simulink model "turbo_controller"  (R2025a)
settings: Solver=FixedStepAuto  StartTime=0.0  StopTime=inf  FixedStep=0.001  RelTol=1e-3
PostLoadFcn:
  | % 自动定位同目录CubeMX文件；不需要外部初始化脚本。
  | codertarget.data.setParameterValue('turbo_controller','STM32CubeMX.ProjectFile',fullfile(fileparts(get_param('turbo_controller','FileName')),'turbo_f407.ioc'));
InitFcn:
  | % 中文说明：按原控制器字段与类型创建三组接口总线；控制参数已内嵌。
  | tc_names=["EValve_Cycle" "EValve_Open" "Eblast_Cycle" "Eblast_Open" "Motor_Cycle" "Motor_Open" "EValve_Enable" "Eblast_Enable" "Motor_Enable" "SWO_Firework" "SWO_BleedAir" "EngineState" "Flag_ECUReset_Clear" "Flag_ECUReset_Save" "Flag_Reset_Enable" "Accelerator" "Nc_dem" "Nc"]; tc_types=["uint16" "uint16" "uint16" "uint16" "uint16" "uint16" "uint8" "uint8" "uint8" "uint8" "uint8" "uint8" "uint8" "uint8" "uint8" "single" "single" "single"];
  | for tc_k=1:numel(tc_names)
  |  tc_e(tc_k)=Simulink.BusElement; tc_e(tc_k).Name=char(tc_names(tc_k)); tc_e(tc_k).DataType=char(tc_types(tc_k));
  | end
  | EngineControl_Out=Simulink.Bus; EngineControl_Out.DataScope='Exported'; EngineControl_Out.Elements=tc_e;
  | clear tc_e tc_names tc_types tc_k
  | tc_names=["savedata1" "savedata2" "savedata3" "savedata4" "savedata5" "savedata6" "savedata7" "savedata8" "savedata9" "savedata10" "savedata11" "savedata12" "savedata13" "savedata14" "savedata15" "savedata16" "savedata17" "savedata18" "savedata19" "savedata20" "savedata21" "savedata22" "savedata23" "savedata24" "savedata25"]; tc_types=["single" "single" "single" "single" "single" "single" "single" "single" "single" "single" "single" "single" "single" "single" "single" "single" "single" "single" "single" "single" "single" "single" "single" "single" "single"];
  | for tc_k=1:numel(tc_names)
  |  tc_e(tc_k)=Simulink.BusElement; tc_e(tc_k).Name=char(tc_names(tc_k)); tc_e(tc_k).DataType=char(tc_types(tc_k));
  | end
  | SaveData_Out=Simulink.Bus; SaveData_Out.DataScope='Exported'; SaveData_Out.Elements=tc_e;
  | clear tc_e tc_names tc_types tc_k
  | tc_names=["senddata1" "senddata2" "senddata3" "senddata4" "senddata5" "senddata6" "senddata7" "senddata8" "senddata9" "senddata10" "senddata11" "senddata12" "senddata13" "senddata14" "senddata15" "senddata16" "senddata17" "senddata18" "senddata19" "senddata20" "senddata21" "senddata22" "senddata23" "senddata24" "senddata25" "senddata26" "senddata27" "senddata28" "senddata29"]; tc_types=["uint8" "uint8" "uint8" "uint8" "uint8" "uint8" "uint8" "uint8" "uint8" "uint8" "uint8" "uint8" "uint8" "uint8" "uint8" "uint8" "uint8" "uint8" "uint8" "uint8" "uint8" "uint8" "uint8" "uint8" "uint8" "uint8" "uint8" "uint8" "uint8"];
  | for tc_k=1:numel(tc_names)
  |  tc_e(tc_k)=Simulink.BusElement; tc_e(tc_k).Name=char(tc_names(tc_k)); tc_e(tc_k).DataType=char(tc_types(tc_k));
  | end
  | SendData_Out=Simulink.Bus; SendData_Out.DataScope='Exported'; SendData_Out.Elements=tc_e;
  | clear tc_e tc_names tc_types tc_k
  | 
  | % 以下为接口中文说明；只设置描述，不改变数值或数据类型。
  | EngineControl_Out.Description='执行控制输出（阀、电机、点火、状态及复位请求）';
  | tc_cn=["EValve_Cycle（主油阀周期计数（每计数2毫秒））" "EValve_Open（主油阀开通计数（每计数2毫秒））" "Eblast_Cycle（副油阀周期计数（每计数2毫秒））" "Eblast_Open（副油阀开通计数（每计数2毫秒））" "Motor_Cycle（起动电机周期计数）" "Motor_Open（起动电机开通计数）" "EValve_Enable（主油阀驱动使能）" "Eblast_Enable（副油阀驱动使能）" "Motor_Enable（起动电机使能）" "SWO_Firework（点火器使能（1开））" "SWO_BleedAir（引气阀使能（1开））" "EngineState（发动机状态）" "Flag_ECUReset_Clear（清除复位恢复状态请求）" "Flag_ECUReset_Save（保存复位恢复数据请求）" "Flag_Reset_Enable（处理器软件复位请求）" "Accelerator（油门／油泵给定控制量）" "Nc_dem（控制目标转速）" "Nc（发动机反馈转速（转每分））"];
  | tc_elements=EngineControl_Out.Elements;
  | for tc_k=1:numel(tc_cn)
  |  tc_elements(tc_k).Description=char(tc_cn(tc_k));
  | end
  | EngineControl_Out.Elements=tc_elements;
  | clear tc_cn tc_elements tc_k
  | SaveData_Out.Description='25项运行记录；字段含义按当前模型数据来源解释';
  | tc_cn=["savedata1（指令回显记录）" "savedata2（入口总温记录（℃））" "savedata3（电源电压记录）" "savedata4（排气温度记录（℃））" "savedata5（标定燃油压力记录）" "savedata6（副油阀占空比记录（％））" "savedata7（主油阀占空比记录（％））" "savedata8（温度修正转速记录）" "savedata9（开关输出及反馈位域）" "savedata10（物理转速记录）" "savedata11（油泵目标给定原始值）" "savedata12（起动电机占空比记录（％））" "savedata13（发动机状态码记录）" "savedata14（故障告警位域记录）" "savedata15（模型记录帧序号）" "savedata16（处理器温度记录（℃））" "savedata17（装订转速记录（沿用旧电源字段名））" "savedata18（导航高度记录）" "savedata19（飞行空速记录）" "savedata20（主阀旧记录位（恒零保留））" "savedata21（第21项保留记录（恒零））" "savedata22（保留记录项22）" "savedata23（保留记录项23）" "savedata24（保留记录项24）" "savedata25（保留记录项25）"];
  | tc_elements=SaveData_Out.Elements;
  | for tc_k=1:numel(tc_cn)
  |  tc_elements(tc_k).Description=char(tc_cn(tc_k));
  | end
  | SaveData_Out.Elements=tc_elements;
  | clear tc_cn tc_elements tc_k
  | SendData_Out.Description='29字段回传及外设命令接口；板端上位机帧只取第3至27字段';
  | tc_cn=["senddata1（回传发送允许标志（不直接上线路））" "senddata2（回传载荷长度25字节）" "senddata3（回传指令回显字节）" "senddata4（总温编码字节（℃＋80））" "senddata5（电源电压编码字节）" "senddata6（排温编码高字节）" "senddata7（排温编码低字节）" "senddata8（燃油压力编码高字节）" "senddata9（燃油压力编码低字节）" "senddata10（副油阀占空比字节（％））" "senddata11（主油阀占空比字节（％））" "senddata12（修正转速编码高字节）" "senddata13（修正转速编码低字节）" "senddata14（驱动及反馈状态位域）" "senddata15（物理转速编码高字节）" "senddata16（物理转速编码低字节）" "senddata17（油泵目标给定高字节（串口二使用））" "senddata18（油泵目标给定低字节（串口二使用））" "senddata19（起动电机占空比命令（串口一使用））" "senddata20（发动机状态码字节）" "senddata21（故障告警位域字节）" "senddata22（帧序号占位（板端另行填写））" "senddata23（处理器温度编码（℃＋50））" "senddata24（控制目标转速编码高字节）" "senddata25（控制目标转速编码低字节）" "senddata26（占位字节（板端改填实测泵速高字节））" "senddata27（占位字节（板端改填实测泵速低字节））" "senddata28（装订转速高字节（本板未发送））" "senddata29（装订转速低字节（本板未发送））"];
  | tc_elements=SendData_Out.Elements;
  | for tc_k=1:numel(tc_cn)
  |  tc_elements(tc_k).Description=char(tc_cn(tc_k));
  | end
  | SendData_Out.Elements=tc_elements;
  | clear tc_cn tc_elements tc_k
  | 
  | 
  | % FRAM模块化事务：接口类型和上电初始状态，随模型保存，无外部初始化文件。
  | clear FM_elements
  | FM_elements(1)=Simulink.BusElement;FM_elements(1).Name='phase';FM_elements(1).DataType='uint8';FM_elements(1).Dimensions=[1 1];FM_elements(1).Description='phase（当前事务阶段）';
  | FM_elements(2)=Simulink.BusElement;FM_elements(2).Name='a';FM_elements(2).DataType='uint8';FM_elements(2).Dimensions=[64 1];FM_elements(2).Description='a（启动时缓存的首区64字节）';
  | FM_elements(3)=Simulink.BusElement;FM_elements(3).Name='active';FM_elements(3).DataType='uint16';FM_elements(3).Dimensions=[1 1];FM_elements(3).Description='active（当前有效记录区地址）';
  | FM_elements(4)=Simulink.BusElement;FM_elements(4).Name='generation';FM_elements(4).DataType='uint32';FM_elements(4).Dimensions=[1 1];FM_elements(4).Description='generation（当前有效记录代号）';
  | FM_elements(5)=Simulink.BusElement;FM_elements(5).Name='record';FM_elements(5).DataType='uint8';FM_elements(5).Dimensions=[64 1];FM_elements(5).Description='record（本次冻结的待写记录）';
  | FM_elements(6)=Simulink.BusElement;FM_elements(6).Name='addr';FM_elements(6).DataType='uint16';FM_elements(6).Dimensions=[1 1];FM_elements(6).Description='addr（本次备用写入地址）';
  | FM_elements(7)=Simulink.BusElement;FM_elements(7).Name='lastSave';FM_elements(7).DataType='single';FM_elements(7).Dimensions=[1 1];FM_elements(7).Description='lastSave（上次开始保存的秒数）';
  | FM_elements(8)=Simulink.BusElement;FM_elements(8).Name='lastState';FM_elements(8).DataType='uint8';FM_elements(8).Dimensions=[1 1];FM_elements(8).Description='lastState（上次保存时的发动机状态）';
  | FM_elements(9)=Simulink.BusElement;FM_elements(9).Name='boot';FM_elements(9).DataType='boolean';FM_elements(9).Dimensions=[1 1];FM_elements(9).Description='boot（启动记录是否允许恢复）';
  | FM_elements(10)=Simulink.BusElement;FM_elements(10).Name='consumed';FM_elements(10).DataType='boolean';FM_elements(10).Dimensions=[1 1];FM_elements(10).Description='consumed（本次启动恢复通知是否已发送）';
  | FM_elements(11)=Simulink.BusElement;FM_elements(11).Name='payload';FM_elements(11).DataType='uint8';FM_elements(11).Dimensions=[20 1];FM_elements(11).Description='payload（当前20字节恢复内容）';
  | ... (+35 lines)
model workspace (MAT data in the model file):
  CRC16_Table_Reference = [0 4129 8258 12387 16516 20645 24774 28903 33032 37161 41290 45419 ... (256 elements, 256x1)]
  PE_Kaer = [0.15402 0.15402 0.12264 0.10076 0.09481 0.07601 0.07111 0.0569 0.05198 0.04926 0.05308 0.04325 ... (13 elements, 1x13)]
  PE_Nr = [21.2982 61.4260372 67.7475458 72.7394382 76.845934 80.6988798 83.8449282 86.6491912 88.9382406 89.178606 91.1938214 93.4068058 ... (13 elements, 1x13)]
  PE_Pump_Translate = 33.5999984741
  PE_RotaSpeed_Translate = 860
  PE_Taer = [0.4939154 0.4939154 0.40780982 0.34066978 0.31622756 0.30405716 0.34300244 0.26785022 0.37393554 0.23914836 0.44563948 0.31044662 ... (13 elements, 1x13)]
  PF_ACCFULLRANGE = 3360
  PF_Flag_ECUReset = 0
  PF_Flag_rx_suc = 1
  PF_Gear_Info = [40000; 45000; 50000; 55000; 57000; 59000; 60000; 61000; 61000; 61000; 61000; 61000]
  PF_K_TiaoJie = 1
  PF_Kpu = 10
  PF_MySet_Rxdata = [0 0 0 0 0 0 0 0 0 0 0 0 ... (50 elements, 50x1)]
  PF_MyUsart1_Rxdata = [0 0 0 0 0 0 0 0 0 0 0 0 ... (50 elements, 50x1)]
  PF_MyUsart2_Rxdata = [0 0 0 0 0 0 0 0 0 0 0 0 ... (50 elements, 50x1)]
  PF_Reset_Information = [0 0 0 0 0 0 0 0 0 0 0 0 ... (20 elements, 20x1)]
  PF_Sensor_X1_T4 = [0 4095]
  PF_Sensor_X2_T4 = [0 1.66666698456]
  PF_Sensor_X3_T4 = [0 504 999 1497 2010 2529 3051 3568 4076 4571 4959]
  PF_Sensor_X_P2 = [0.5 3]
  PF_Sensor_X_Poil = [0.5 3]
  PF_Sensor_X_T1t = [-50 300]
  PF_Sensor_X_Vpower = [0 3]
  PF_Sensor_X_Vpump = [0 3]
  PF_Sensor_Y1_T4 = [0 3]
  PF_Sensor_Y2_T4 = [0 5000]
  PF_Sensor_Y3_T4 = [0 100 200 300 400 500 600 700 800 900 980]
  PF_Sensor_Y_P2 = [0 1000]
  PF_Sensor_Y_Poil = [0 1000]
  PF_Sensor_Y_T1t = [-50 300]
  PF_Sensor_Y_Vpower = [0 33]
  PF_Sensor_Y_Vpump = [0 33]
  PG_CtrlMode_CloseLoop : mpt.Parameter (value not decoded)
  PG_CtrlMode_ManualAcc : mpt.Parameter (value not decoded)
  PG_CtrlMode_Origin : mpt.Parameter (value not decoded)
  PG_CtrlMode_Start : mpt.Parameter (value not decoded)
  PG_CtrlMode_Stop : mpt.Parameter (value not decoded)
  PG_ES_Clp : mpt.Parameter (value not decoded)
  PG_ES_EngStart : mpt.Parameter (value not decoded)
  PG_ES_Manual : mpt.Parameter (value not decoded)
  PG_ES_Origin : mpt.Parameter (value not decoded)
  PG_ES_Stop : mpt.Parameter (value not decoded)
  PG_Instr_BleedAirSet : mpt.Parameter (value not decoded)
  PG_Instr_CloseLoop : mpt.Parameter (value not decoded)
  PG_Instr_ECUReSet : mpt.Parameter (value not decoded)
  PG_Instr_EValveSet : mpt.Parameter (value not decoded)
  PG_Instr_EblastSet : mpt.Parameter (value not decoded)
  PG_Instr_Erase : mpt.Parameter (value not decoded)
  PG_Instr_FireWorkSet : mpt.Parameter (value not decoded)
  PG_Instr_ManualPlus : mpt.Parameter (value not decoded)
  PG_Instr_ManualrReduce : mpt.Parameter (value not decoded)
  PG_Instr_MotorSet : mpt.Parameter (value not decoded)
  PG_Instr_OilSet : mpt.Parameter (value not decoded)
  PG_Instr_SelfCheck : mpt.Parameter (value not decoded)
  PG_Instr_Start : mpt.Parameter (value not decoded)
  PG_Instr_Stop : mpt.Parameter (value not decoded)
  PG_Instr_StopZero : Simulink.Parameter (value not decoded)
  PG_Location_Air : Simulink.Parameter (value not decoded)
  PG_Location_Gnd : Simulink.Parameter (value not decoded)
  PG_ServoCtrlMode_CloseLoop : Simulink.Parameter (value not decoded)
  PG_ServoCtrlMode_CloseLoopMax : Simulink.Parameter (value not decoded)
  PG_ServoCtrlMode_CloseLoopMin : Simulink.Parameter (value not decoded)
  PG_ServoCtrlMode_ManualAcc : Simulink.Parameter (value not decoded)
  PG_ServoCtrlMode_ManualAccMax : Simulink.Parameter (value not decoded)
  PG_ServoCtrlMode_ManualAccMin : Simulink.Parameter (value not decoded)
  PG_SpeedDot_Permit : Simulink.Parameter (value not decoded)
  PL_EngineModel_Actuator = [0 10 100]
  PL_EngineModel_EngineStar_Press_P2 = [1013 1098.4 1099.144828 1099.931034 1103.613793 1162.662069 1143.793103 1131.006897 1123.186207 1117.6 1114 1111.806897 ... (127 elements, 1x127)]
  PL_EngineModel_EngineStar_RotaSpeed = [200 2000 9584 9660 10220 10240 10260 10288 10308 10368 10380 10408 ... (127 elements, 1x127)]
  PL_EngineModel_EngineStar_Temp_Exhaust = [128 129 129.1 130 131 131.1 132 133 134 134.1 135 135.1 ... (127 elements, 1x127)]
  PL_EngineModel_EngineStar_Time = [0.05 0.1 0.15 0.2 0.25 0.3 0.35 0.4 0.45 0.5 0.55 0.6 ... (127 elements, 1x127)]
  PL_EngineModel_IdleAbove_Nr = [0 21.2982 61.4260372 67.7475458 72.7394382 76.845934 80.6988798 83.8449282 86.6491912 88.9382406 89.178606 91.1938214 ... (14 elements, 1x14)]
  PL_EngineModel_IdleAbove_P2r = [0.986923266716 1.57907722675 1.81593881076 1.99358499877 2.23044658278 2.43770046879 2.65482358747 2.84233900814 3.03972366149 3.18776215149 3.25684678016 3.3950160375 ... (14 elements, 1x14)]
  PL_EngineModel_IdleAbove_Tempr = [0.0536001429337 1.07200285867 1.63301768805 1.63659103091 1.66875111667 1.72592460247 1.77595140254 1.86171163123 1.95461854565 2.03323208862 2.03323208862 2.13685903162 ... (14 elements, 1x14)]
  PL_EngineModel_IdleAbove_Ter = [0.42434128 0.42434128 0.42434128 0.30669408 0.23570008 0.22150128 0.1997974 0.23803274 0.16115638 0.24279948 0.13600422 0.31308354 ... (14 elements, 1x14)]
  PL_EngineModel_IdleAbove_Wfr = [0 10.142 23.8337 27.8905 31.9473 36.0041 40.0609 44.1177 48.1745 52.2313 52.7384 56.7952 ... (14 elements, 1x14)]
  PL_EngineModel_Press_P2 = [400 400 400 400 400 400 400 400 400 400]
  PL_EngineModel_Rotaspeed = [0 20000 96400]
  PL_EngineModel_Temp_Exhaust = [500 500 500 500 500 500 500 500 500 500]
  PL_Kaer = [0.1 0.1 0.1 0.1 0.1 0.1]
  PL_Nr = [50 60 70 80 90 100]
  PL_Taer = [0.1 0.1 0.1 0.1 0.1 0.1]
  Sig : Simulink.Signal (value not decoded)
  Ts_ms : Simulink.Parameter (value not decoded)
  false : Simulink.Parameter (value not decoded)
  true : Simulink.Parameter (value not decoded)
symbols that are objects in the model workspace (value not decoded): PG_CtrlMode_CloseLoop, PG_CtrlMode_ManualAcc, PG_CtrlMode_Origin, PG_CtrlMode_Start, PG_CtrlMode_Stop, PG_ES_Clp, PG_ES_EngStart, PG_ES_Manual, PG_ES_Origin, PG_ES_Stop, PG_Instr_BleedAirSet, PG_Instr_CloseLoop, PG_Instr_EblastSet, PG_Instr_ECUReSet, PG_Instr_Erase, PG_Instr_EValveSet, PG_Instr_FireWorkSet, PG_Instr_ManualPlus, PG_Instr_ManualrReduce, PG_Instr_MotorSet, PG_Instr_OilSet, PG_Instr_SelfCheck, PG_Instr_Start, PG_Instr_Stop, PG_Instr_StopZero, PG_ServoCtrlMode_CloseLoop, PG_ServoCtrlMode_CloseLoopMax, PG_ServoCtrlMode_CloseLoopMin, PG_ServoCtrlMode_ManualAcc, PG_ServoCtrlMode_ManualAccMax, PG_ServoCtrlMode_ManualAccMin, Ts_ms
libraries: simulink x97, stm32blockslib x10, stm32f4xxblockslib x8
(part 6 of 26)

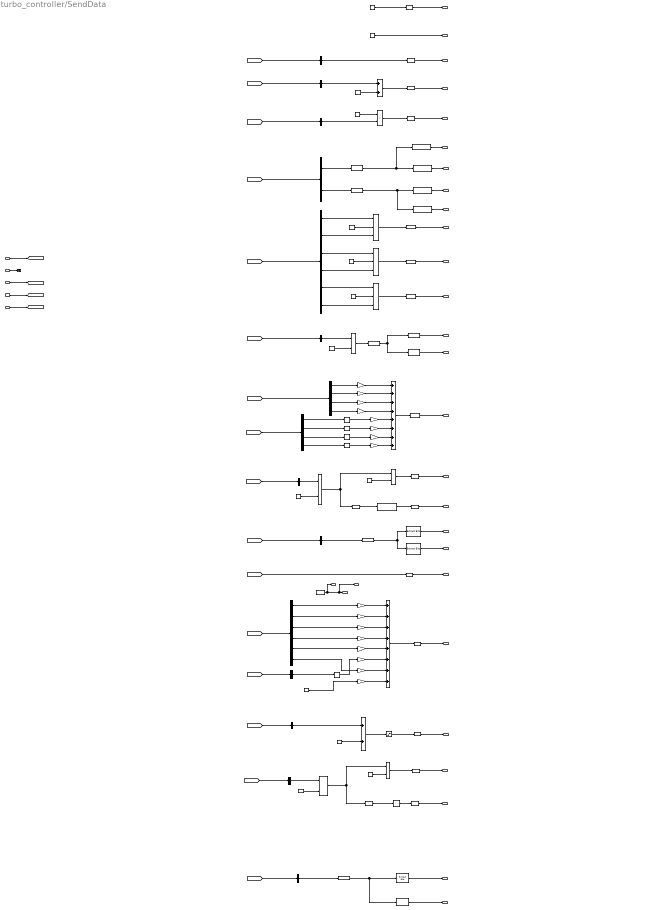
== system turbo_controller/SendData ==
  note: SendData做什么：把运行量编码成回传字段
      |
      | 本页接收传感器/通信总线、执行控制总线、发动机模式和监视告警，把它们变成回传所需的字节编码
      | 。它不直接发送UART，也不在这里生成20 ms发送节拍。
      |
      | 29个输出端口不等于29字节串口帧：端口1是回传使能；端口2是旧协议长度常数25；端口3～27为本页
      | 提供的25个内容字段。后级Payload用AA、55、01作帧头，将端口3～27映射到帧第4～28字节，并覆盖
      | 第23、27、28字节；再追加两项校验，才形成30字节发送帧。
      |
      | 端口28、29虽然叫NBumpH/L，在本页实际由COMM.SpeedLoad拆字节，不能称作实测泵速。真实泵速来自
      | Out01_Pump，在后级直接覆盖帧第27、28字节。
      |
      | S_SDM当前接Unused_SDM终止端，不参与这些内容。端口名字中的H/L表示高/低字节，编码值必须按下
      | 文比例还原，不能全部直接当作物理量。
  note: 温度、供电和油压怎样编码
      |
      | T0取Sensor.T0，先加80再向下取整转uint8：编码=floor(T0+80)。例25 ℃回传105，上位机减80还原
      | 。这里不是ADC原始计数，温度标定已在ISM完成。
      |
      | 处理器温度取Sensor.Tecu：先加50，再限制0～255，最后向下取整转uint8。例25 ℃得到75；超出范
      | 围会截住，上位机减50只能得到截断后的温度。
      |
      | 供电取Sensor.Vpower：编码=floor(5×电压)，例24 V得到120，解码时除5。这是ADC换算电压，不是CO
      | MM.V_Power字段。
      |
      | T4取Sensor.T4_Filter，POil取Sensor.POil_Filter：各先向下取整转uint16，再拆成高低字节，没有
      | 在本页额外乘10。例排温500对应高1、低244；接收端按高×256+低还原500。油压单位沿用传感器标定
      | ，不能仅凭POil名称写成kPa。
  note: 三类转速与泵给定，不能混作一项
      |
      | 物理转速取Sensor.Origin_Nc，先除2；高字节=floor((转速/2)/256)，低字节=floor(转速/2) AND 25
      | 5。
      |
      | 温度修正转速取Sensor.HuanSuanZhuanSu，先除2并向下取整为uint16，再拆高低字节。它是修正后的
      | 量，不是原始脉冲计数。
      |
      | 目标转速取COMM.SpeedLoad，也先除2，再取高低字节。例目标50000 rpm，编码25000，高97、低168；
      | 上位机合成后乘2还原50000。三条转速通道的编码步长均为2 rpm，奇数或小数部分会损失。
      |
      | NBump_MuBiaoH/L实际取执行总线Accelerator，直接转uint16并拆字节，不除2。例泵给定3000对应高1
      | 1、低184。它是控制编码，不是泵转速实测值。
      |
      | 本页NBumpH/L取COMM.SpeedLoad直接转uint16拆分：50000会得到高195、低80。此旧接口不用于代表当
      | 前实测泵速；最终帧泵速位置由Telemetry覆盖。
  note: 主阀、副阀和电机：回传开通比例
      |
      | 读取执行控制总线中的Open和Cycle，分别计算：
      | 主油阀编码=floor(100×EValve_Open/EValve_Cycle)；
      | 副油阀编码=floor(100×Eblast_Open/Eblast_Cycle)；
      | 电机编码=floor(100×Motor_Open/Motor_Cycle)。
      |
      | 例阀门周期30、开通15，得到50，表示50%的开通比例；不是开阀15 ms，也不是50%的机械位置。电机
      | 周期100、开通40得到40。
      |
      | 这些量来自驱动设定，不是阀门位置传感器或实测转速。是否使能还要看开关量字段；不能只看比例非
      | 0就断言硬件正在工作。
      |
      | 本页按原计算直接相除，没有额外在此分支添加分母保护。上游应给出正常周期值；本次只更新说明，
      | 不调整算法。
  note: 开关量字节：低四位命令，高四位反馈取反
      |
      | KaiGuanLiang把8个布尔量乘1、2、4、8、16、32、64、128后相加。位0是最低位。
      |
      | 位0（1）：SWO_Firework点火使能；
      | 位1（2）：EValve_Enable主阀使能；
      | 位2（4）：Eblast_Enable副阀使能；
      | 位3（8）：SWO_BleedAir引气使能；
      | 位4（16）：NOT SWI_Firework；
      | 位5（32）：NOT SWI_EValve；
      | 位6（64）：NOT SWI_Eblast；
      | 位7（128）：NOT SWI_BleedAir。
      |
      | 低四位取执行命令，高四位取传感器反馈的逻辑反值。不能把两组都解释成命令，也不能跳过NOT直接
      | 按原GPIO电平解释。
      |
      | 例只有主阀使能和取反后的主阀反馈为真，字节为2+32=34。解码某位可用bitand(字节,该位权重)是否
      | 非0。这里未打包Motor_Enable，电机比例另走Motor端口。
  note: 告警字节与发动机模式
      |
      | GuZhangXingXi同样按位权相加：
      | 位0（1）：Alarm_OverTemp；
      | 位1（2）：Alarm_OverSpeed；
      | 位2（4）：Flag_NcFailure；
      | 位3（8）：Alarm_ECUReset；
      | 位4（16）：Alarm_Vpower_Low；
      | 位5（32）：NOT Sensor.SWI_ValveErr；
      | 位6（64）：Lock_NcFailure；
      | 位7（128）：当前常量0。
      |
      | 例如超温和欠压同时为真，其他位为假，得到1+16=17。位5明确使用反馈取反，不能只写“阀门故障”
      | 却省略它与原反馈的反向关系。
      |
      | FaDongJiZhuangTai直接将EngineState转uint8：0初始、1普通起动、2闭环、3手动、4停车。它不是上
      | 位机指令编号，也不是起动图A～F阶段。此处只编码，不触发告警或模式转换。
  note: 输出端口1～15分别是什么
      |
      | 1 ChuanShuBiaoZhi：固定1，供后级判断回传允许。
      | 2 ShuJuChangDu：旧协议常数25；不是最终UART发送长度。
      | 3 ZhiLingHuiChuan：COMM.Instr_XianShi转uint8。
      | 4 T0：入口温度加80的单字节编码。
      | 5 dianyuandianya：电压乘5的单字节编码。
      | 6/7 T4_H/L：排温整数高/低字节。
      | 8/9 POil_H/L：油压标定整数高/低字节。
      | 10 Eblast：副油阀开通比例百分数。
      | 11 EValve：主油阀开通比例百分数。
      | 12/13 HuanSuanZhuanSuH/L：修正转速除2后拆字节。
      | 14 KaiGuanLiang：执行开关与取反反馈的位组合。
      | 15 WuLiZhuanSuH1：物理转速除2后的高字节。
      |
      | 本页编号是Outport序号。后级串口帧前面还有AA、55、01，因此端口3进入帧第4字节，而不是帧第3字
      | 节。
  note: 输出端口16～29及后级覆盖关系
      |
      | 16 WuLiZhuanSuL1：物理转速除2后的低字节。
      | 17/18 NBump_MuBiaoH/L：Accelerator泵给定高/低字节。
      | 19 Motor：电机开通比例百分数。
      | 20 FaDongJiZhuangTai：发动机运行模式编号。
      | 21 GuZhangXingXi：告警位组合。
      | 22 rt：本页固定0占位；后级帧第23字节改为循环帧号。
      | 23 TECU：处理器温度加50、限幅后的编码。
      | 24/25 MuBiaoZhuanSuH2/L2：目标转速除2后拆字节。
      | 26 QW、27 ER：本页固定0保留值；最终帧对应位置被真实泵速高、低字节覆盖。
      | 28/29 NBumpH/L：本页由SpeedLoad直接拆出的旧接口，不是实测泵速；Payload映射只取senddata1及3
      | ～27。
      |
      | 最终泵反馈填入帧第27/28字节，来源为Out01_Pump滤波结果；帧第23字节由FrameCounter覆盖；最后
      | 第29/30字节是累加与异或校验。SendData自身不生成这些最终覆盖值和校验。
  note: 读图时注意：编码精度与拆字节
      |
      | 高低字节合成：整数=高字节×256+低字节。
      | 拆分16位整数：高=floor(整数/256)，低=整数 AND 255。例1000拆为3和232，不能按十进制把它拆成1
      | 0和00。
      |
      | 本页多数转换采用Floor，即向下取整。uint8仅容纳0～255，uint16容纳0～65535；除TECU已有限幅和
      | 饱和处理外，不能把每处类型转换都理解为会自动截到上下限。正常工作范围外可能发生回绕，本次未
      | 修改这些设置。
      |
      | 比例、偏置和两字节编码都是协议表示方式，不是新的传感器标定。回传目标、执行命令、测量反馈的
      | 含义不同；判断最终线上数据还要继续看BoardOutput/Out03_Telemetry的覆盖和校验。
  S_SPM : Inport
      settings: AttributesFormatString=S_SPM（通信及传感器信息总线）
  S_SDM : Inport  Port=2
      settings: AttributesFormatString=S_SDM（传感器自检与状态数据）
  S_Servo_Out : Inport  Port=3
      settings: AttributesFormatString=S_Servo_Out（伺服输出）
  S_EngineState : Inport  Port=4
      settings: AttributesFormatString=S_EngineState（发动机状态）
  S_MAlarm : Inport  Port=5
      settings: AttributesFormatString=S_MAlarm（报警）
  Bitwise Operator2 : simulink/Logic and Bit Operations/Bitwise Operator  logicop=AND  UseBitMask=on  BitMask=bin2dec('11111111')  BitMaskRealWorld=Stored Integer
      settings: AttributesFormatString=Bitwise Operator2（按位运算运算2）
  Bitwise Operator3 : simulink/Logic and Bit Operations/Bitwise Operator  logicop=AND  UseBitMask=on  BitMask=bin2dec('11111111')  BitMaskRealWorld=Stored Integer
      settings: AttributesFormatString=Bitwise Operator3（按位运算运算3）
  Bus Selector1 : BusSelector  OutputSignals=Sensor（传感器信息总线）.T0（入口总温）
      settings: AttributesFormatString=Bus Selector1（总线选择器1）
  Bus Selector10 : BusSelector  OutputSignals=EValve_Open（主油阀开通计数）,EValve_Cycle（主油阀周期计数）,Eblast_Open（副油阀开通计数）,Eblast_Cycle（副油阀周期计数）,Motor_Open（起动电机开通计数）,Motor_Cycle（起动电机周期计数）
      settings: AttributesFormatString=Bus Selector10（总线选择器10）
  Bus Selector11 : BusSelector  OutputSignals=SWO_Firework（点火器使能）,EValve_Enable（主油阀使能）,Eblast_Enable（副油阀使能）,SWO_BleedAir（引气阀使能）
      settings: AttributesFormatString=Bus Selector11（总线选择器11）
  Bus Selector12 : BusSelector  OutputSignals=Sensor（传感器信息总线）.Tecu（处理器温度）
      settings: AttributesFormatString=Bus Selector12（总线选择器12）
  Bus Selector13 : BusSelector  OutputSignals=COMM（通信信息总线）.Instr_XianShi（指令回显）
      settings: AttributesFormatString=Bus Selector13（总线选择器13）
  Bus Selector14 : BusSelector  OutputSignals=Sensor（传感器信息总线）.SWI_Firework（点火器告警反馈）,Sensor（传感器信息总线）.SWI_EValve（主油阀反馈）,Sensor（传感器信息总线）.SWI_Eblast（副油阀反馈）,Sensor（传感器信息总线）.SWI_BleedAir（引气阀反馈）
      settings: AttributesFormatString=Bus Selector14（总线选择器14）
  Bus Selector15 : BusSelector  OutputSignals=Accelerator（油泵给定控制量）
      settings: AttributesFormatString=Bus Selector15（总线选择器15）
  Bus Selector16 : BusSelector  OutputSignals=COMM（通信信息总线）.SpeedLoad（装订转速）
      settings: AttributesFormatString=Bus Selector16（总线选择器16）
  Bus Selector17 : BusSelector  OutputSignals=Sensor（传感器信息总线）.HuanSuanZhuanSu（温度修正转速）
      settings: AttributesFormatString=Bus Selector17（总线选择器17）
  Bus Selector18 : BusSelector  OutputSignals=Sensor（传感器信息总线）.SWI_ValveErr（阀门综合告警反馈）
      settings: AttributesFormatString=Bus Selector18（总线选择器18）
  Bus Selector2 : BusSelector  OutputSignals=Sensor（传感器信息总线）.T4_Filter（滤波后排气温度）,Sensor（传感器信息总线）.POil_Filter（滤波后燃油压力）
      settings: AttributesFormatString=Bus Selector2（总线选择器2）
  Bus Selector3 : BusSelector  OutputSignals=Sensor（传感器信息总线）.Vpower（电源电压）
      settings: AttributesFormatString=Bus Selector3（总线选择器3）
  Bus Selector4 : BusSelector  OutputSignals=Sensor（传感器信息总线）.Origin_Nc（原位转速）
      settings: AttributesFormatString=Bus Selector4（总线选择器4）
  Bus Selector8 : BusSelector  OutputSignals=COMM（通信信息总线）.SpeedLoad（装订转速）
      settings: AttributesFormatString=Bus Selector8（总线选择器8）
  Bus Selector9 : BusSelector  OutputSignals=Alarm_OverTemp（超温告警）,Alarm_OverSpeed（超转告警）,Flag_NcFailure（转速传感器故障标志）,Alarm_ECUReset（控制器复位告警）,Alarm_Vpower_Low（电源欠压告警）,Lock_NcFailure（转速故障锁存）
      settings: AttributesFormatString=Bus Selector9（总线选择器9）
  Data Type Conversion1 : DataTypeConversion  OutDataTypeStr=uint32  SaturateOnIntegerOverflow=off  RndMeth=Floor
      settings: AttributesFormatString=Data Type Conversion1（数据类型转换1）
  Data Type Conversion11 : DataTypeConversion  OutDataTypeStr=uint8  RndMeth=Floor
      settings: AttributesFormatString=Data Type Conversion11（数据类型转换11）
  Data Type Conversion{4..5,9,12..13,15..20,22..24} (14 alike) : DataTypeConversion  OutDataTypeStr=uint8  SaturateOnIntegerOverflow=off  RndMeth=Floor
      Data Type Conversion12 settings: AttributesFormatString=Data Type Conversion12（数据类型转换12）
      Data Type Conversion13 settings: AttributesFormatString=Data Type Conversion13（数据类型转换13）
      Data Type Conversion15 settings: AttributesFormatString=Data Type Conversion15（数据类型转换15）
      Data Type Conversion16 settings: AttributesFormatString=Data Type Conversion16（数据类型转换16）
      Data Type Conversion17 settings: AttributesFormatString=Data Type Conversion17（数据类型转换17）
      Data Type Conversion18 settings: AttributesFormatString=Data Type Conversion18（数据类型转换18）
      Data Type Conversion19 settings: AttributesFormatString=Data Type Conversion19（数据类型转换19）
      Data Type Conversion20 settings: AttributesFormatString=Data Type Conversion20（数据类型转换20）
      Data Type Conversion22 settings: AttributesFormatString=Data Type Conversion22（数据类型转换22）
      Data Type Conversion23 settings: AttributesFormatString=Data Type Conversion23（数据类型转换23）
      Data Type Conversion24 settings: AttributesFormatString=Data Type Conversion24（数据类型转换24）
      Data Type Conversion4 settings: AttributesFormatString=Data Type Conversion4（数据类型转换4）
      Data Type Conversion5 settings: AttributesFormatString=Data Type Conversion5（数据类型转换5）
      Data Type Conversion9 settings: AttributesFormatString=Data Type Conversion9（数据类型转换9）
  Data Type Conversion{6..8,25..26} (5 alike) : DataTypeConversion  OutDataTypeStr=uint16  SaturateOnIntegerOverflow=off  RndMeth=Floor
      Data Type Conversion25 settings: AttributesFormatString=Data Type Conversion25（数据类型转换25）
      Data Type Conversion26 settings: AttributesFormatString=Data Type Conversion26（数据类型转换26）
      Data Type Conversion6 settings: AttributesFormatString=Data Type Conversion6（数据类型转换6）
      Data Type Conversion7 settings: AttributesFormatString=Data Type Conversion7（数据类型转换7）
      Data Type Conversion8 settings: AttributesFormatString=Data Type Conversion8（数据类型转换8）
  Data Type Conversion3 : DataTypeConversion  OutDataTypeStr=uint32  SaturateOnIntegerOverflow=off  RndMeth=Floor
      settings: AttributesFormatString=Data Type Conversion3（数据类型转换3）
  Extract Bits1 : simulink/Logic and Bit Operations/Extract Bits  Description=|  bitsToExtract=Range of bits  numBits=8  bitIdxRange=[8 15]  outScalingMode=Treat bit field as an integer
      | Extract Bits1：从整数编码中取出指定二进制位
      | 
      | 当前选择Range of bits，位范围[8 15]，输出按整数解释。位号从0开始，0是最低位。它不是按十进制字符截取，也不改变传感器标定。
      | 
      | 取高8位：结果=floor(原整数/256) mod 256。例如1000（十六进制03E8）取出3。
      | 
      | 用于回传拆字节时，高低字节要按协议顺序发送；接收方按“高×256+低”才能还原原整数。
      settings: AttributesFormatString=Extract Bits1（提取位1）
  Extract Bits10 : simulink/Logic and Bit Operations/Extract Bits  Description=|  bitsToExtract=Range of bits  numBits=8  bitIdxRange=[0 7]  outScalingMode=Treat bit field as an integer
      | Extract Bits10：从整数编码中取出指定二进制位
      | 
      | 当前选择Range of bits，位范围[0 7]，输出按整数解释。位号从0开始，0是最低位。它不是按十进制字符截取，也不改变传感器标定。
      | 
      | 取低8位：结果=原整数 mod 256。例如1000（十六进制03E8）取出232。
      | 
      | 用于回传拆字节时，高低字节要按协议顺序发送；接收方按“高×256+低”才能还原原整数。
      settings: AttributesFormatString=Extract Bits10（提取位10）
  Extract Bits2 : simulink/Logic and Bit Operations/Extract Bits  Description=|  bitsToExtract=Range of bits  numBits=8  bitIdxRange=[8 15]  outScalingMode=Treat bit field as an integer
      | Extract Bits2：从整数编码中取出指定二进制位
      | 
      | 当前选择Range of bits，位范围[8 15]，输出按整数解释。位号从0开始，0是最低位。它不是按十进制字符截取，也不改变传感器标定。
      | 
      | 取高8位：结果=floor(原整数/256) mod 256。例如1000（十六进制03E8）取出3。
      | 
      | 用于回传拆字节时，高低字节要按协议顺序发送；接收方按“高×256+低”才能还原原整数。
      settings: AttributesFormatString=Extract Bits2（提取位2）
  Extract Bits3 : simulink/Logic and Bit Operations/Extract Bits  Description=|  bitsToExtract=Range of bits  numBits=8  bitIdxRange=[0 7]  outScalingMode=Treat bit field as an integer
      | Extract Bits3：从整数编码中取出指定二进制位
      | 
      | 当前选择Range of bits，位范围[0 7]，输出按整数解释。位号从0开始，0是最低位。它不是按十进制字符截取，也不改变传感器标定。
      | 
      | 取低8位：结果=原整数 mod 256。例如1000（十六进制03E8）取出232。
      | 
      | 用于回传拆字节时，高低字节要按协议顺序发送；接收方按“高×256+低”才能还原原整数。
      settings: AttributesFormatString=Extract Bits3（提取位3）
  Extract Bits4 : simulink/Logic and Bit Operations/Extract Bits  Description=|  bitsToExtract=Range of bits  numBits=8  bitIdxRange=[8 15]  outScalingMode=Treat bit field as an integer
      | Extract Bits4：从整数编码中取出指定二进制位
      | 
      | 当前选择Range of bits，位范围[8 15]，输出按整数解释。位号从0开始，0是最低位。它不是按十进制字符截取，也不改变传感器标定。
      | 
      | 取高8位：结果=floor(原整数/256) mod 256。例如1000（十六进制03E8）取出3。
      | 
      | 用于回传拆字节时，高低字节要按协议顺序发送；接收方按“高×256+低”才能还原原整数。
      settings: AttributesFormatString=Extract Bits4（提取位4）
  Extract Bits5 : simulink/Logic and Bit Operations/Extract Bits  Description=|  bitsToExtract=Range of bits  numBits=8  bitIdxRange=[0 7]  outScalingMode=Treat bit field as an integer
      | Extract Bits5：从整数编码中取出指定二进制位
      | 
      | 当前选择Range of bits，位范围[0 7]，输出按整数解释。位号从0开始，0是最低位。它不是按十进制字符截取，也不改变传感器标定。
      | 
      | 取低8位：结果=原整数 mod 256。例如1000（十六进制03E8）取出232。
      | 
      | 用于回传拆字节时，高低字节要按协议顺序发送；接收方按“高×256+低”才能还原原整数。
      settings: AttributesFormatString=Extract Bits5（提取位5）
  Extract Bits6 : simulink/Logic and Bit Operations/Extract Bits  Description=|  bitsToExtract=Range of bits  numBits=8  bitIdxRange=[0 7]  outScalingMode=Treat bit field as an integer
      | Extract Bits6：从整数编码中取出指定二进制位
      | 
      | 当前选择Range of bits，位范围[0 7]，输出按整数解释。位号从0开始，0是最低位。它不是按十进制字符截取，也不改变传感器标定。
      | 
      | 取低8位：结果=原整数 mod 256。例如1000（十六进制03E8）取出232。
      | 
      | 用于回传拆字节时，高低字节要按协议顺序发送；接收方按“高×256+低”才能还原原整数。
      settings: AttributesFormatString=Extract Bits6（提取位6）
  Extract Bits7 : simulink/Logic and Bit Operations/Extract Bits  Description=|  bitsToExtract=Range of bits  numBits=8  bitIdxRange=[8 15]  outScalingMode=Treat bit field as an integer
      | Extract Bits7：从整数编码中取出指定二进制位
      | 
      | 当前选择Range of bits，位范围[8 15]，输出按整数解释。位号从0开始，0是最低位。它不是按十进制字符截取，也不改变传感器标定。
      | 
      | 取高8位：结果=floor(原整数/256) mod 256。例如1000（十六进制03E8）取出3。
      | 
      | 用于回传拆字节时，高低字节要按协议顺序发送；接收方按“高×256+低”才能还原原整数。
      settings: AttributesFormatString=Extract Bits7（提取位7）
  Extract Bits8 : simulink/Logic and Bit Operations/Extract Bits  Description=|  bitsToExtract=Range of bits  numBits=8  bitIdxRange=[0 7]  outScalingMode=Treat bit field as an integer
      | Extract Bits8：从整数编码中取出指定二进制位
      | 
      | 当前选择Range of bits，位范围[0 7]，输出按整数解释。位号从0开始，0是最低位。它不是按十进制字符截取，也不改变传感器标定。
      | 
      | 取低8位：结果=原整数 mod 256。例如1000（十六进制03E8）取出232。
      | 
      | 用于回传拆字节时，高低字节要按协议顺序发送；接收方按“高×256+低”才能还原原整数。
      settings: AttributesFormatString=Extract Bits8（提取位8）
  Extract Bits9 : simulink/Logic and Bit Operations/Extract Bits  Description=|  bitsToExtract=Range of bits  numBits=8  bitIdxRange=[8 15]  outScalingMode=Treat bit field as an integer
      | Extract Bits9：从整数编码中取出指定二进制位
      | 
      | 当前选择Range of bits，位范围[8 15]，输出按整数解释。位号从0开始，0是最低位。它不是按十进制字符截取，也不改变传感器标定。
      | 
      | 取高8位：结果=floor(原整数/256) mod 256。例如1000（十六进制03E8）取出3。
      | 
      | 用于回传拆字节时，高低字节要按协议顺序发送；接收方按“高×256+低”才能还原原整数。
      settings: AttributesFormatString=Extract Bits9（提取位9）
  Gain1 : Gain  OutDataTypeStr=uint8
      settings: AttributesFormatString=Gain1（乘以系数1）
  Gain10 : Gain  Gain=16  OutDataTypeStr=uint8
      settings: AttributesFormatString=Gain10（乘以系数16）
  Gain11 : Gain  Gain=32  OutDataTypeStr=uint8
      settings: AttributesFormatString=Gain11（乘以系数32）
  Gain12 : Gain  Gain=64  OutDataTypeStr=uint8
      settings: AttributesFormatString=Gain12（乘以系数64）
  Gain13 : Gain  Gain=128  OutDataTypeStr=uint8
      settings: AttributesFormatString=Gain13（乘以系数128）
  Gain14 : Gain  Gain=2  OutDataTypeStr=uint8
      settings: AttributesFormatString=Gain14（乘以系数2）
  Gain15 : Gain  Gain=4  OutDataTypeStr=uint8
      settings: AttributesFormatString=Gain15（乘以系数4）
  Gain16 : Gain  Gain=8  OutDataTypeStr=uint8
      settings: AttributesFormatString=Gain16（乘以系数8）
  Gain2 : Gain  Gain=16  OutDataTypeStr=uint8
      settings: AttributesFormatString=Gain2（乘以系数16）
  Gain3 : Gain  Gain=32  OutDataTypeStr=uint8
      settings: AttributesFormatString=Gain3（乘以系数32）
  Gain4 : Gain  Gain=64  OutDataTypeStr=uint8
      settings: AttributesFormatString=Gain4（乘以系数64）
  Gain5 : Gain  Gain=128  OutDataTypeStr=uint8
      settings: AttributesFormatString=Gain5（乘以系数128）
  Gain6 : Gain  Gain=2  OutDataTypeStr=uint8
      settings: AttributesFormatString=Gain6（乘以系数2）
  Gain7 : Gain  Gain=4  OutDataTypeStr=uint8
      settings: AttributesFormatString=Gain7（乘以系数4）
  Gain8 : Gain  Gain=8  OutDataTypeStr=uint8
      settings: AttributesFormatString=Gain8（乘以系数8）
  Gain9 : Gain  OutDataTypeStr=uint8
      settings: AttributesFormatString=Gain9（乘以系数1）
  Logical Operator{,1..4} (5 alike) : Logic  Operator=NOT  AllPortsSameDT=off  OutDataTypeStr=boolean
      Logical Operator settings: AttributesFormatString=Logical Operator（逻辑运算）
      Logical Operator1 settings: AttributesFormatString=Logical Operator1（逻辑运算1）
      Logical Operator2 settings: AttributesFormatString=Logical Operator2（逻辑运算2）
      Logical Operator3 settings: AttributesFormatString=Logical Operator3（逻辑运算3）
      Logical Operator4 settings: AttributesFormatString=Logical Operator4（逻辑运算4）
  Product{1..2,4,10..11} (5 alike) : Product  Inputs=*/
      Product1 settings: AttributesFormatString=Product1（乘法1）
      Product10 settings: AttributesFormatString=Product10（乘法10）
      Product11 settings: AttributesFormatString=Product11（乘法11）
      Product2 settings: AttributesFormatString=Product2（乘法2）
      Product4 settings: AttributesFormatString=Product4（乘法4）
  Product19 : Product  Inputs=**
      settings: AttributesFormatString=Product19（乘法19）
  Product3 : Product  Inputs=**/
      settings: AttributesFormatString=Product3（乘法3）
  Product7 : Product  Inputs=**/
      settings: AttributesFormatString=Product7（乘法7）
  Product8 : Product  Inputs=**/
      settings: AttributesFormatString=Product8（乘法8）
  ReservedByte_Zero : Constant  Value=uint8(0)  OutDataTypeStr=uint8
  Sum of Elements1 : Sum  Inputs=++++++++
      settings: AttributesFormatString=Sum of Elements1（加法求和的元素1）
  Sum of Elements2 : Sum
      settings: AttributesFormatString=Sum of Elements2（加法求和的元素2）
  Sum of Elements4 : Sum  Inputs=++++++++
      settings: AttributesFormatString=Sum of Elements4（加法求和的元素4）
  Sum of Elements5 : Sum
      settings: AttributesFormatString=Sum of Elements5（加法求和的元素5）
  TECU_ByteRange : Saturate  Description=处理器温度回传编码 Tecu + 50 的可表示字节范围。低于 0 输出 0，高于 255 输出 255；范围内保持原编码。  UpperLimit=single(255)  LowerLimit=single(0)
  Unused_SDM : Terminator
  dth = T0-288.10 : Constant  Value=0  OutDataTypeStr=single  SampleTime=-1
      settings: AttributesFormatString=dth = T0-288.10（固定常量0（旧名称不参与计算））
  dth = T0-288.11 : Constant  OutDataTypeStr=uint8  SampleTime=-1
      settings: AttributesFormatString=dth = T0-288.11（固定常量1（旧名称不参与计算））
  dth = T0-288.12 : Constant  Value=100  OutDataTypeStr=single  SampleTime=-1
      settings: AttributesFormatString=dth = T0-288.12（固定常量100（旧名称不参与计算））
  dth = T0-288.13 : Constant  Value=100  OutDataTypeStr=single  SampleTime=-1
      settings: AttributesFormatString=dth = T0-288.13（固定常量100（旧名称不参与计算））
  dth = T0-288.2 : Constant  Value=2  OutDataTypeStr=single  SampleTime=-1
      settings: AttributesFormatString=dth = T0-288.2（固定常量2（旧名称不参与计算））
  dth = T0-288.20 : Constant  Value=50  OutDataTypeStr=single  SampleTime=-1
      settings: AttributesFormatString=dth = T0-288.20（固定常量50（旧名称不参与计算））
  dth = T0-288.29 : Constant  Value=256  OutDataTypeStr=single  SampleTime=-1
      settings: AttributesFormatString=dth = T0-288.29（固定常量256（旧名称不参与计算））
  dth = T0-288.3 : Constant  Value=5  OutDataTypeStr=single  SampleTime=-1
      settings: AttributesFormatString=dth = T0-288.3（固定常量5（旧名称不参与计算））
  dth = T0-288.30 : Constant  Value=2  OutDataTypeStr=single  SampleTime=-1
      settings: AttributesFormatString=dth = T0-288.30（固定常量2（旧名称不参与计算））
  dth = T0-288.38 : Constant  Value=25  OutDataTypeStr=uint8  SampleTime=-1
      settings: AttributesFormatString=dth = T0-288.38（固定常量25（旧名称不参与计算））
  dth = T0-288.4 : Constant  Value=256  OutDataTypeStr=single  SampleTime=-1
      settings: AttributesFormatString=dth = T0-288.4（固定常量256（旧名称不参与计算））
  dth = T0-288.5 : Constant  Value=2  OutDataTypeStr=single  SampleTime=-1
      settings: AttributesFormatString=dth = T0-288.5（固定常量2（旧名称不参与计算））
  dth = T0-288.6 : Constant  Value=80  OutDataTypeStr=single  SampleTime=-1
      settings: AttributesFormatString=dth = T0-288.6（固定常量80（旧名称不参与计算））
  dth = T0-288.9 : Constant  Value=100  OutDataTypeStr=single  SampleTime=-1
      settings: AttributesFormatString=dth = T0-288.9（固定常量100（旧名称不参与计算））
  ChuanShuBiaoZhi : Outport  Description=输出端口1 ChuanShuBiaoZhi：回传使能常量1。
      settings: AttributesFormatString=ChuanShuBiaoZhi（回传发送允许标志（不直接上线路））
  ShuJuChangDu : Outport  Description=输出端口2 ShuJuChangDu：旧协议长度常量25，不是最终30字节发送长度。  Port=2
      settings: AttributesFormatString=ShuJuChangDu（回传载荷长度25字节）
  ZhiLingHuiChuan : Outport  Description=输出端口3 ZhiLingHuiChuan：指令回显COMM.Instr_XianShi。  Port=3
      settings: AttributesFormatString=ZhiLingHuiChuan（回传指令回显字节）
  T0 : Outport  Description=输出端口4 T0：入口温度编码=floor(T0+80)。  Port=4
      settings: AttributesFormatString=T0（总温编码字节（℃＋80））
  dianyuandianya : Outport  Description=输出端口5 dianyuandianya：供电编码=floor(Vpower×5)。  Port=5
      settings: AttributesFormatString=dianyuandianya（电源电压编码字节）
  T4_H : Outport  Description=输出端口6 T4_H：滤波排温整数的高字节。  Port=6
      settings: AttributesFormatString=T4_H（排温编码高字节）
  T4_L : Outport  Description=输出端口7 T4_L：滤波排温整数的低字节。  Port=7
      settings: AttributesFormatString=T4_L（排温编码低字节）
  POil_H : Outport  Description=输出端口8 POil_H：滤波油压整数的高字节。  Port=8
      settings: AttributesFormatString=POil_H（燃油压力编码高字节）
  POil_L : Outport  Description=输出端口9 POil_L：滤波油压整数的低字节。  Port=9
      settings: AttributesFormatString=POil_L（燃油压力编码低字节）
  Eblast : Outport  Description=输出端口10 Eblast：副阀开通比例百分数。  Port=10
      settings: AttributesFormatString=Eblast（副油阀占空比字节（％））
  EValve : Outport  Description=输出端口11 EValve：主阀开通比例百分数。  Port=11
      settings: AttributesFormatString=EValve（主油阀占空比字节（％））
  HuanSuanZhuanSuH : Outport  Description=输出端口12 HuanSuanZhuanSuH：修正转速除2后的高字节。  Port=12
      settings: AttributesFormatString=HuanSuanZhuanSuH（修正转速编码高字节）
  HuanSuanZhuanSuL : Outport  Description=输出端口13 HuanSuanZhuanSuL：修正转速除2后的低字节。  Port=13
      settings: AttributesFormatString=HuanSuanZhuanSuL（修正转速编码低字节）
  KaiGuanLiang : Outport  Description=输出端口14 KaiGuanLiang：低四位命令、高四位反馈取反组合。  Port=14
      settings: AttributesFormatString=KaiGuanLiang（驱动及反馈状态位域）
  WuLiZhuanSuH1 : Outport  Description=输出端口15 WuLiZhuanSuH1：物理转速除2后的高字节。  Port=15
      settings: AttributesFormatString=WuLiZhuanSuH1（物理转速编码高字节）
  WuLiZhuanSuL1 : Outport  Description=输出端口16 WuLiZhuanSuL1：物理转速除2后的低字节。  Port=16
      settings: AttributesFormatString=WuLiZhuanSuL1（物理转速编码低字节）
  NBump_MuBiaoH : Outport  Description=输出端口17 NBump_MuBiaoH：Accelerator泵给定直接拆分的高字节。  Port=17
      settings: AttributesFormatString=NBump_MuBiaoH（油泵目标给定高字节（串口二使用））
  NBump_MuBiaoL : Outport  Description=输出端口18 NBump_MuBiaoL：Accelerator泵给定直接拆分的低字节。  Port=18
      settings: AttributesFormatString=NBump_MuBiaoL（油泵目标给定低字节（串口二使用））
  Motor : Outport  Description=输出端口19 Motor：电机开通比例百分数。  Port=19
      settings: AttributesFormatString=Motor（起动电机占空比命令（串口一使用））
  FaDongJiZhuangTai : Outport  Description=输出端口20 FaDongJiZhuangTai：EngineState模式0初始1普通起动2闭环3手动4停车。  Port=20
      settings: AttributesFormatString=FaDongJiZhuangTai（发动机状态码字节）
  GuZhangXingXi : Outport  Description=输出端口21 GuZhangXingXi：按位组合告警，位5为NOT SWI_ValveErr。  Port=21
      settings: AttributesFormatString=GuZhangXingXi（故障告警位域字节）
  rt : Outport  Description=输出端口22 rt：帧号占位常量0；后级帧第23字节覆盖。  Port=22  OutDataTypeStr=uint8
  TECU : Outport  Description=输出端口23 TECU：处理器温度加50并限制0～255后向下取整。  Port=23
      settings: AttributesFormatString=TECU（处理器温度编码（℃＋50））
  MuBiaoiZhuanSuH2 : Outport  Description=输出端口24 MuBiaoiZhuanSuH2：SpeedLoad目标转速除2后的高字节。  Port=24
      settings: AttributesFormatString=MuBiaoiZhuanSuH2（控制目标转速编码高字节）
  MuBiaoZhuanSuL2 : Outport  Description=输出端口25 MuBiaoZhuanSuL2：SpeedLoad目标转速除2后的低字节。  Port=25
      settings: AttributesFormatString=MuBiaoZhuanSuL2（控制目标转速编码低字节）
  QW : Outport  Description=输出端口26 QW：保留0；最终帧第27字节被真实泵速高字节覆盖。  Port=26
      settings: AttributesFormatString=QW（占位字节（板端改填实测泵速高字节））
  ER : Outport  Description=输出端口27 ER：保留0；最终帧第28字节被真实泵速低字节覆盖。  Port=27
      settings: AttributesFormatString=ER（占位字节（板端改填实测泵速低字节））
  NBumpH : Outport  Description=输出端口28 NBumpH：SpeedLoad直接拆分高字节；不是实测泵速。  Port=28
      settings: AttributesFormatString=NBumpH（装订转速高字节（本板未发送））
  NBumpL : Outport  Description=输出端口29 NBumpL：SpeedLoad直接拆分低字节；不是实测泵速。  Port=29
      settings: AttributesFormatString=NBumpL（装订转速低字节（本板未发送））
  wires:
  S_SPM/1 -> [S_SPM]
  S_Servo_Out/1 -> [S_Servo_Out]
  S_MAlarm/1 -> [MAlarm]
  S_EngineState/1 -> [EngineState]
  Bus Selector12/1 -> Sum of Elements2/1  "<Tecu（处理器温度）>"
  [MAlarm] -> Bus Selector9/1
  Data Type Conversion16/1 -> GuZhangXingXi/1
  Sum of Elements1/1 -> Data Type Conversion16/1
  [S_SPM] -> Bus Selector12/1
  dth = T0-288.38/1 -> ShuJuChangDu/1
  Data Type Conversion18/1 -> ChuanShuBiaoZhi/1
  [S_SPM] -> Bus Selector13/1
  dth = T0-288.11/1 -> Data Type Conversion18/1
  [S_SPM] -> Bus Selector1/1
  Bus Selector1/1 -> Sum of Elements5/1  "<T0（入口总温）>"
  [S_SPM] -> Bus Selector2/1
  Bus Selector2/1 -> Data Type Conversion7/1  "<T4_Filter（滤波后排气温度）>"
  Data Type Conversion7/1 -> Extract Bits6/1, Extract Bits2/1
  Extract Bits2/1 -> T4_H/1
  Extract Bits6/1 -> T4_L/1
  Bus Selector2/2 -> Data Type Conversion8/1  "<POil_Filter（滤波后燃油压力）>"
  Data Type Conversion8/1 -> Extract Bits5/1, Extract Bits4/1
  Extract Bits4/1 -> POil_H/1
  Extract Bits5/1 -> POil_L/1
  Bus Selector3/1 -> Product19/2  "<Vpower（电源电压）>"
  [S_SPM] -> Bus Selector3/1
  Product3/1 -> Data Type Conversion20/1
  Product7/1 -> Data Type Conversion22/1
  Product8/1 -> Data Type Conversion23/1
  [S_SPM] -> Bus Selector4/1
  Bitwise Operator2/1 -> Data Type Conversion9/1
  Data Type Conversion9/1 -> WuLiZhuanSuL1/1
  Product11/1 -> Data Type Conversion12/1
  dth = T0-288.29/1 -> Product11/2
  Data Type Conversion12/1 -> WuLiZhuanSuH1/1
  Bus Selector4/1 -> Product10/1  "<Origin_Nc（原位转速）>"
  Data Type Conversion1/1 -> Bitwise Operator2/1
  dth = T0-288.30/1 -> Product10/2
  Product10/1 -> Product11/1, Data Type Conversion1/1
  [EngineState] -> Data Type Conversion13/1
  [S_SPM] -> Bus Selector8/1
  Bitwise Operator3/1 -> Data Type Conversion17/1
  Data Type Conversion17/1 -> MuBiaoZhuanSuL2/1
  Product2/1 -> Data Type Conversion15/1
  dth = T0-288.4/1 -> Product2/2
  Data Type Conversion15/1 -> MuBiaoiZhuanSuH2/1
  Bus Selector8/1 -> Product1/1  "<SpeedLoad（装订转速）>"
  Data Type Conversion3/1 -> Bitwise Operator3/1
  dth = T0-288.5/1 -> Product1/2
  Product1/1 -> Data Type Conversion3/1, Product2/1
  Data Type Conversion19/1 -> ZhiLingHuiChuan/1
  Bus Selector13/1 -> Data Type Conversion19/1  "<Instr_XianShi（指令回显）>"
  [S_Servo_Out] -> Bus Selector10/1
  Bus Selector10/2 -> Product3/3  "<EValve_Cycle（主油阀周期计数）>"
  dth = T0-288.13/1 -> Product3/2
  Bus Selector10/1 -> Product3/1  "<EValve_Open（主油阀开通计数）>"
  Data Type Conversion20/1 -> EValve/1
  Data Type Conversion22/1 -> Eblast/1
  Data Type Conversion23/1 -> Motor/1
  Bus Selector10/4 -> Product7/3  "<Eblast_Cycle（副油阀周期计数）>"
  dth = T0-288.9/1 -> Product7/2
  Bus Selector10/3 -> Product7/1  "<Eblast_Open（副油阀开通计数）>"
  Bus Selector10/6 -> Product8/3  "<Motor_Cycle（起动电机周期计数）>"
  dth = T0-288.12/1 -> Product8/2
  Bus Selector10/5 -> Product8/1  "<Motor_Open（起动电机开通计数）>"
  dth = T0-288.20/1 -> Sum of Elements2/2
  [S_SPM] -> Bus Selector14/1
  Bus Selector14/1 -> Logical Operator/1  "<SWI_Firework（点火器告警反馈）>"
  Bus Selector14/4 -> Logical Operator3/1  "<SWI_BleedAir（引气阀反馈）>"
  Bus Selector14/2 -> Logical Operator1/1  "<SWI_EValve（主油阀反馈）>"
  Bus Selector14/3 -> Logical Operator2/1  "<SWI_Eblast（副油阀反馈）>"
  Sum of Elements4/1 -> Data Type Conversion24/1
  Logical Operator/1 -> Gain2/1
  Logical Operator1/1 -> Gain3/1
  Logical Operator2/1 -> Gain4/1
  Logical Operator3/1 -> Gain5/1
  [S_SPM] -> Bus Selector16/1
  Data Type Conversion26/1 -> Extract Bits7/1, Extract Bits8/1
  Bus Selector16/1 -> Data Type Conversion26/1  "<SpeedLoad（装订转速）>"
  Extract Bits8/1 -> NBumpL/1
  Extract Bits7/1 -> NBumpH/1
  [S_Servo_Out] -> Bus Selector15/1
  Data Type Conversion25/1 -> Extract Bits1/1, Extract Bits3/1
  Bus Selector15/1 -> Data Type Conversion25/1  "<Accelerator（油泵给定控制量）>"
  Extract Bits1/1 -> NBump_MuBiaoH/1
  Extract Bits3/1 -> NBump_MuBiaoL/1
  [S_Servo_Out] -> Bus Selector11/1
  Data Type Conversion24/1 -> KaiGuanLiang/1
  Data Type Conversion4/1 -> dianyuandianya/1
  dth = T0-288.3/1 -> Product19/1
  Product19/1 -> Data Type Conversion4/1
  Data Type Conversion5/1 -> T0/1
  dth = T0-288.6/1 -> Sum of Elements5/2
  Sum of Elements5/1 -> Data Type Conversion5/1
  Gain1/1 -> Sum of Elements4/1
  Gain6/1 -> Sum of Elements4/2
  Gain7/1 -> Sum of Elements4/3
  Gain8/1 -> Sum of Elements4/4
  Gain2/1 -> Sum of Elements4/5
  Gain3/1 -> Sum of Elements4/6
  Gain4/1 -> Sum of Elements4/7
  Gain5/1 -> Sum of Elements4/8
  Bus Selector11/1 -> Gain1/1  "<SWO_Firework（点火器使能）>"
  Bus Selector11/2 -> Gain6/1  "<EValve_Enable（主油阀使能）>"
  Bus Selector11/3 -> Gain7/1  "<Eblast_Enable（副油阀使能）>"
  Bus Selector11/4 -> Gain8/1  "<SWO_BleedAir（引气阀使能）>"
  [S_SPM] -> Bus Selector17/1
  Bus Selector17/1 -> Product4/1  "<HuanSuanZhuanSu（温度修正转速）>"
  dth = T0-288.2/1 -> Product4/2
  Product4/1 -> Data Type Conversion6/1
  Data Type Conversion6/1 -> Extract Bits10/1, Extract Bits9/1
  Extract Bits9/1 -> HuanSuanZhuanSuH/1
  Extract Bits10/1 -> HuanSuanZhuanSuL/1
  Gain9/1 -> Sum of Elements1/1
  Gain14/1 -> Sum of Elements1/2
  Gain15/1 -> Sum of Elements1/3
  Gain16/1 -> Sum of Elements1/4
  Gain10/1 -> Sum of Elements1/5
  Gain11/1 -> Sum of Elements1/6
  Gain12/1 -> Sum of Elements1/7
  Gain13/1 -> Sum of Elements1/8
  Bus Selector9/1 -> Gain9/1  "<Alarm_OverTemp（超温告警）>"
  Bus Selector9/2 -> Gain14/1  "<Alarm_OverSpeed（超转告警）>"
  Bus Selector9/3 -> Gain15/1  "<Flag_NcFailure（转速传感器故障标志）>"
  Bus Selector9/4 -> Gain16/1  "<Alarm_ECUReset（控制器复位告警）>"
  Bus Selector9/5 -> Gain10/1  "<Alarm_Vpower_Low（电源欠压告警）>"
  [S_SPM] -> Bus Selector18/1
  Bus Selector18/1 -> Logical Operator4/1  "<SWI_ValveErr（阀门综合告警反馈）>"
  dth = T0-288.10/1 -> Gain13/1
  Data Type Conversion13/1 -> FaDongJiZhuangTai/1
  Bus Selector9/6 -> Gain12/1  "<Lock_NcFailure（转速故障锁存）>"
  Logical Operator4/1 -> Gain11/1
  ReservedByte_Zero/1 -> ER/1, rt/1, QW/1
  S_SDM/1 -> Unused_SDM/1
  TECU_ByteRange/1 -> Data Type Conversion11/1
  Sum of Elements2/1 -> TECU_ByteRange/1
  Data Type Conversion11/1 -> TECU/1

== system turbo_controller/BoardInput_输入换算与协议解析/In01_Host（上位机命令解析） ==
  note: 从上位机字节流中取出一条可靠命令
      |
      | 串口每次提供一个字节数组和实际接收数量。数组容量不是有效数据长度，必须只处理本次计数范围内
      | 的字节；否则尾部旧数据可能被误当作新命令。
      |
      | Receive按字节顺序调用Collect：先找十六进制AA、55两个帧头，再把后续数据放入14字节缓存。收齐
      | 后交Verify检查累加校验和异或校验。两种校验都一致才接收这帧，失败时不覆盖上次有效命令。
      |
      | 通过的14字节放进原控制算法沿用的50项接口，未用部分补零，并保存“有新命令”等待通知。每20 m
      | s节拍把这次新命令标志交给根层ControlRate；没有新有效帧时仍保留上次内容，但不应把保持内容解
      | 释成又收到一条命令。
      |
      | 输出的命令数组随后进入COMMRead_ISM/CMMRead。那里的Instr_Analyse才把FC等原始命令字节解释成
      | 内部Instr，SpeedLoad_Analyse解析目标转速。因此本层负责可靠收帧，尚未决定发动机该启动还是停
      | 车。
  Rx（串口接收字节）_1 : Inport  OutDataTypeStr=uint8
  Count（有效字节数）_2 : Inport  Port=2  OutDataTypeStr=uint32
  Seconds（当前秒数）_3 : Inport  Port=3  OutDataTypeStr=double
  Constant（常量）_4 : Constant  Value=1000  OutDataTypeStr=double
  Constant（常量）_7 : Constant  Value=20  OutDataTypeStr=double
  Constant（常量）_9 : Constant  Value=0  OutDataTypeStr=double
  Every20ms（20毫秒更新许可）_10 : RelationalOperator  Operator===  OutDataTypeStr=boolean  RndMeth=Simplest  InputSameDT=off
  Format（保持原输出维度）_1 : Reshape
  Milliseconds（秒换算为毫秒）_5 : Product  Inputs=**  SaturateOnIntegerOverflow=on  OutDataTypeStr=Inherit: Same as first input
  Phase20（20毫秒相位）_8 : Math  Operator=mod
  Receive（逐字节组帧与保持有效结果）_108 : Subsystem  Description=|
      | 上位机接收流程：按1→2→3→4阅读，第5步管理通知时机
      | 
      | 这页只保留三个输入、两个输出、一个循环块和五个处理步骤。
      | Rx：接收数组；Count：本批新收到多少字节；ControlTick：20 ms更新许可。
      | Command：最近有效的50项命令；Flag：本次是否通知控制任务有新命令。
      | 
      | Step01取一项字节，决定本项有效及何时结束循环。
      | Step02识别AA55并拼14字节，未拼完的数据保留到下次。
      | Step03检查收齐事件及累加、异或校验，给出本次接受事件。
      | Step04有效才更新命令，否则保持上一条；14字节后补36个0。
      | Step05记住是否有新命令，等20 ms许可时输出通知。
      | 
      | 三种记忆各管一件事：半帧缓存属于Step02；上一条有效命令属于Step04；尚未报告标志属于Step05。候选帧、有效命令、通知标志不能混为一谈。
      | 
      | Loop让这五步在本次调用内逐字节重复，不是五步各等一个采样周期。Step01的下一序号反馈Loop，达到本批数量或64项就结束。因此一批能处理多字节，也能连续接受多帧。
      | 
      | 本次仅拆分层次，保留原来的循环、类型转换、初值、校验与保持逻辑。点开每一步可看具体例子及输入输出含义。
  RoundTime（按原规则取整）_6 : Rounding  Operator=round
  Vector1D（保持原一维向量接口）_2 : Reshape
  Flag（新命令通知）_109 : Outport
  Command（最近有效命令）_110 : Outport  Port=2
  wires:
  Milliseconds（秒换算为毫秒）_5/1 -> RoundTime（按原规则取整）_6/1  "Milliseconds（秒换算为毫秒）"
  Count（有效字节数）_2/1 -> Receive（逐字节组帧与保持有效结果）_108/2(Count（本次有效字节数）_12)  "Count（有效字节数）"
  Seconds（当前秒数）_3/1 -> Milliseconds（秒换算为毫秒）_5/1  "Seconds（当前秒数）"
  Constant（常量）_4/1 -> Milliseconds（秒换算为毫秒）_5/2  "Constant（常量）"
  Phase20（20毫秒相位）_8/1 -> Every20ms（20毫秒更新许可）_10/1  "Phase20（20毫秒相位）"
  RoundTime（按原规则取整）_6/1 -> Phase20（20毫秒相位）_8/1  "RoundTime（按原规则取整）"
  Constant（常量）_7/1 -> Phase20（20毫秒相位）_8/2  "Constant（常量）"
  Constant（常量）_9/1 -> Every20ms（20毫秒更新许可）_10/2  "Constant（常量）"
  Format（保持原输出维度）_1/1 -> Flag（新命令通知）_109/1
  Receive（逐字节组帧与保持有效结果）_108/1(Flag（20毫秒新命令通知）_106) -> Format（保持原输出维度）_1/1  "Receive（逐字节组帧与保持有效结果）"
  Rx（串口接收字节）_1/1 -> Receive（逐字节组帧与保持有效结果）_108/1(Rx（本次接收字节）_11)  "Rx（串口接收字节）"
  Every20ms（20毫秒更新许可）_10/1 -> Receive（逐字节组帧与保持有效结果）_108/3(ControlTick（20毫秒更新许可）_13)  "Every20ms（20毫秒更新许可）"
  Receive（逐字节组帧与保持有效结果）_108/2(Command（最近有效命令）_107) -> Vector1D（保持原一维向量接口）_2/1  "Receive（逐字节组帧与保持有效结果）"
  Vector1D（保持原一维向量接口）_2/1 -> Command（最近有效命令）_110/1

== system turbo_controller/BoardInput_输入换算与协议解析/In02_Motor（电机反馈解析） ==
  note: 电机反馈字节怎样变成转速
      |
      | 输入来自USART1电机串口，包括字节数组和实际有效数量。逐字节识别AA55帧头、收齐9字节后，先核
      | 对CRC16；只有本次新帧通过校验，才采用第6、7字节。
      |
      | 第6项为高字节，第7项为低字节，先合成16位原始数：
      | 原始数 = 第6字节 × 256 + 第7字节；
      | 电机反馈转速 = floor(原始数 / 3)。
      | 例如高字节1、低字节44合成300，除以3后得到100。除3是本工程保留的反馈比例，floor表示向下取整
      | 。
      |
      | 通过校验后更新并记住转速；没有新完整帧或CRC失败时保持上次有效反馈。保持旧值不代表电机这一
      | 毫秒又发来了同样的数据。
      |
      | 结果作为In05_Speed的一种转速来源。上一电机给定非零时，它的优先级高于定时器捕获估算。该模块
      | 是接收解析，不负责发电机控制命令。
  Rx（串口接收字节）_111 : Inport  OutDataTypeStr=uint8
  Count（有效字节数）_112 : Inport  Port=2  OutDataTypeStr=uint32
  Format（保持原输出维度）_1 : Reshape
  Receive（逐字节组帧与保持有效结果）_235 : Subsystem  Description=|
      | 电机反馈接收流程：按1→2→3→4阅读
      | 
      | 第一步只遍历本批有效字节，最多处理64项；第二步识别AA55、收齐9字节，并保存尚未收完的半帧；第三步确认本字节刚收齐且CRC通过；第四步换算数值并保存最近有效结果。
      | 
      | Loop在一次调用内逐字节重复这些步骤，不是每一步各等1 ms。接收数组的Index每批重新遍历，收帧Position可以跨批保留，两者不是同一个位置。
      | 
      | 有效帧第6、7字节合成整数，再除3向下取整得到电机反馈；没有有效新帧时保持旧值。
      | 
      | 本次将原有处理块按职责封装，保留原协议、初始化、数据类型、校验和循环行为。各步骤内部可看输入、公式和例子。
  Speed（反馈转速）_236 : Outport
  wires:
  Count（有效字节数）_112/1 -> Receive（逐字节组帧与保持有效结果）_235/2(Count（本次有效字节数）_114)  "Count（有效字节数）"
  Rx（串口接收字节）_111/1 -> Receive（逐字节组帧与保持有效结果）_235/1(Rx（本次接收字节）_113)  "Rx（串口接收字节）"
  Format（保持原输出维度）_1/1 -> Speed（反馈转速）_236/1
  Receive（逐字节组帧与保持有效结果）_235/1(Speed（当前有效反馈）_234) -> Format（保持原输出维度）_1/1  "Receive（逐字节组帧与保持有效结果）"
